simulink model "test_codegen_sim_03"  (Simulink 7.9)
settings: Solver=ode45  StartTime=0.0  StopTime=10.0  FixedStep=0.1  RelTol=1e-3
libraries: mpt_sim x1
settings Model: Creator=mato  LastModifiedBy=mato
settings SolverCC: AutoInsertRateTranBlk=on

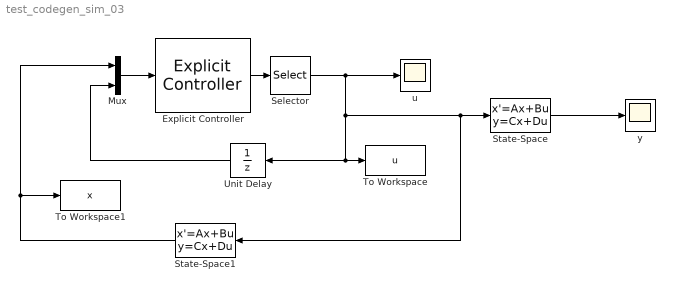
== system test_codegen_sim_03 ==
  Explicit Controller : mpt_sim/Explicit Controller
      link override S-Function: FunctionName=codetest03_sfunc
  Mux : Mux  Inputs=2
  Selector : Selector  InputPortWidth=4  IndexOptions=Index vector (dialog)  Indices=1  OutputSizes=1
  State-Space : StateSpace  A="[ -0.1768   -0.6291   -1.4286;   -2.1321   -1.2038   -0.0209;    1.1454   -0.2539   -0.5607];"  B=[1; 0; 1];  C=[0 -1 1];  D=0  X0=[0;0;0]
  State-Space1 : StateSpace  A="[ -0.1768   -0.6291   -1.4286;   -2.1321   -1.2038   -0.0209;    1.1454   -0.2539   -0.5607];"  B=[1; 0; 1];  C=eye(3)  D=zeros(3,1)  X0=[0;0;0]
  To Workspace : ToWorkspace  VariableName=u  SampleTime=0.1
  To Workspace1 : ToWorkspace  VariableName=x  SampleTime=0.1
  Unit Delay : UnitDelay  SampleTime=-1
  u : Scope
      settings: TimeRange=10
  y : Scope
      settings: TimeRange=10
  wires:
  Explicit Controller/1 -> Selector/1
  State-Space/1 -> y/1
  State-Space1/1 -> To Workspace1/1, Mux/1
  Selector/1 -> u/1, State-Space/1, State-Space1/1, To Workspace/1, Unit Delay/1
  Mux/1 -> Explicit Controller/1
  Unit Delay/1 -> Mux/2
